simulink model "runway_landing_assist"  (R2019a)
settings: Solver=FixedStepDiscrete  StartTime=0.0  StopTime=20  FixedStep=0.1  RelTol=1e-3
settings Model: Creator=ABHI  LastModifiedBy=ABHI

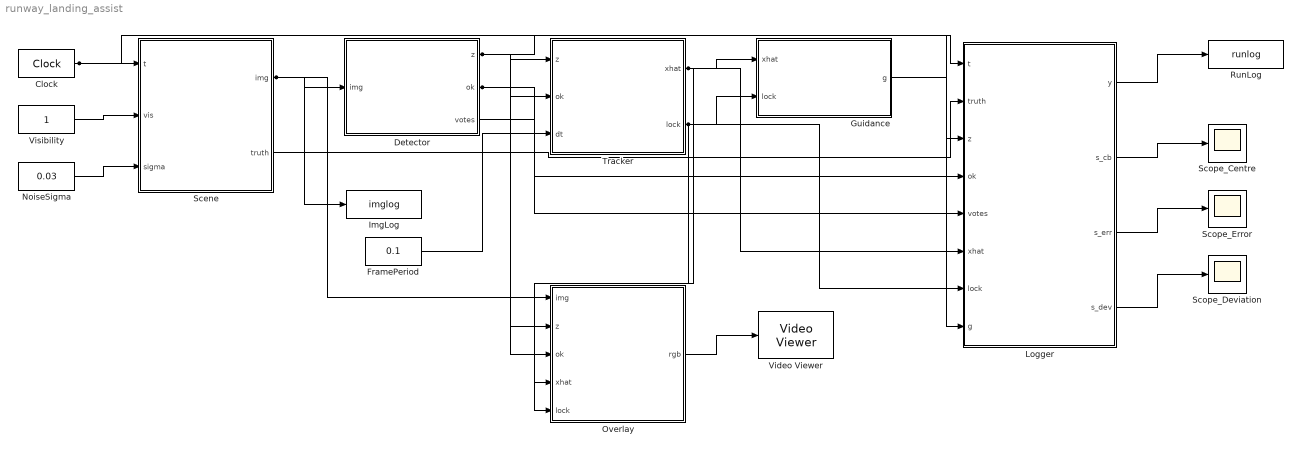
== system runway_landing_assist ==
  Clock : DigitalClock  SampleTime=0.1
  Detector : MATLAB Function  TreatAsAtomicUnit=on
  FramePeriod : Constant  Value=0.1
  Guidance : MATLAB Function  TreatAsAtomicUnit=on
  ImgLog : ToWorkspace  VariableName=imglog  SampleTime=0.1
  Logger : MATLAB Function  TreatAsAtomicUnit=on
  NoiseSigma : Constant  Value=0.03
  Overlay : MATLAB Function  TreatAsAtomicUnit=on
  RunLog : ToWorkspace  VariableName=runlog  SampleTime=0.1
  Scene : MATLAB Function  TreatAsAtomicUnit=on
  Scope_Centre : Scope
  Scope_Deviation : Scope
  Scope_Error : Scope
  Tracker : MATLAB Function  TreatAsAtomicUnit=on
  Video Viewer : VideoViewer  FigPos=[2041 741 418 304]
  Visibility : Constant
  wires:
  Clock/1 -> Scene/1(t), Logger/1(t)
  Visibility/1 -> Scene/2(vis)
  NoiseSigma/1 -> Scene/3(sigma)
  Scene/1(img) -> Detector/1(img), ImgLog/1, Overlay/1(img)
  Detector/1(z) -> Tracker/1(z), Overlay/2(z), Logger/3(z)
  Detector/2(ok) -> Tracker/2(ok), Overlay/3(ok), Logger/4(ok)
  FramePeriod/1 -> Tracker/3(dt)
  Tracker/1(xhat) -> Guidance/1(xhat), Overlay/4(xhat), Logger/6(xhat)
  Tracker/2(lock) -> Guidance/2(lock), Overlay/5(lock), Logger/7(lock)
  Overlay/1(rgb) -> Video Viewer/1
  Scene/2(truth) -> Logger/2(truth)
  Detector/3(votes) -> Logger/5(votes)
  Guidance/1(g) -> Logger/8(g)
  Logger/1(y) -> RunLog/1
  Logger/2(s_cb) -> Scope_Centre/1
  Logger/3(s_err) -> Scope_Error/1
  Logger/4(s_dev) -> Scope_Deviation/1

== matlab function runway_landing_assist/Detector ==
  data: img input; z output; ok output; votes output
function [z, ok, votes] = fcn(img)
%#codegen
[z, ok, votes] = runway_detect(img);

== matlab function runway_landing_assist/Scene ==
  data: t input; img output; vis input; sigma input; truth output
function [img, truth] = fcn(t, vis, sigma)
%#codegen
[img, truth] = runway_scene(t, vis, sigma);

== matlab function runway_landing_assist/Tracker ==
  data: z input; xhat output; ok input; dt input; lock output
function [xhat, lock] = fcn(z, ok, dt)
%#codegen
[xhat, lock] = runway_tracker(z, ok, dt);

== matlab function runway_landing_assist/Guidance ==
  data: xhat input; g output; lock input
function g = fcn(xhat, lock)
%#codegen
g = runway_guidance(xhat, lock);

== matlab function runway_landing_assist/Overlay ==
  data: img input; rgb output; z input; ok input; xhat input; lock input
function rgb = fcn(img, z, ok, xhat, lock)
%#codegen
rgb = runway_overlay(img, z, ok, xhat, lock);

== matlab function runway_landing_assist/Logger ==
  data: t input; y output; truth input; z input; ok input; votes input; xhat input; lock input; g input; s_cb output; s_err output; s_dev output
function [y, s_cb, s_err, s_dev] = fcn(t, truth, z, ok, votes, xhat, lock, g)
%#codegen
[y, s_cb, s_err, s_dev] = runway_logger(t, truth, z, ok, votes, xhat, lock, g);
